simulink model "SoH_MPC_SolarPump"  (R2025b)
settings: Solver=ode4  StartTime=0.0  StopTime=86400  FixedStep=5  RelTol=1e-3
values from neighbouring files (symbols this model uses):
  P =     [robustness_same_min_tight.mat]    (also in robustness_same_min_wide.mat; run_day.m = rmfield(P, 'solverStep'); run_fixed_min.m = P0; P.strategy = 3; P.SoH0 = cases{k,2}; solver15_stress_check.m = mpc_params; P.strategy = strategy)
settings Model: Creator=Santhosh  LastModifiedBy=Santhosh

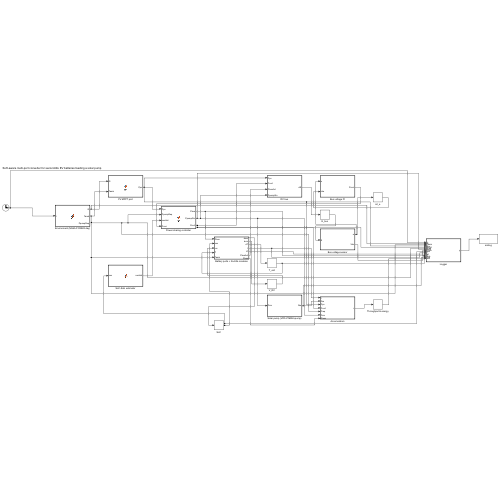
[thumbnail: Simulink's stored preview of the top-level diagram]
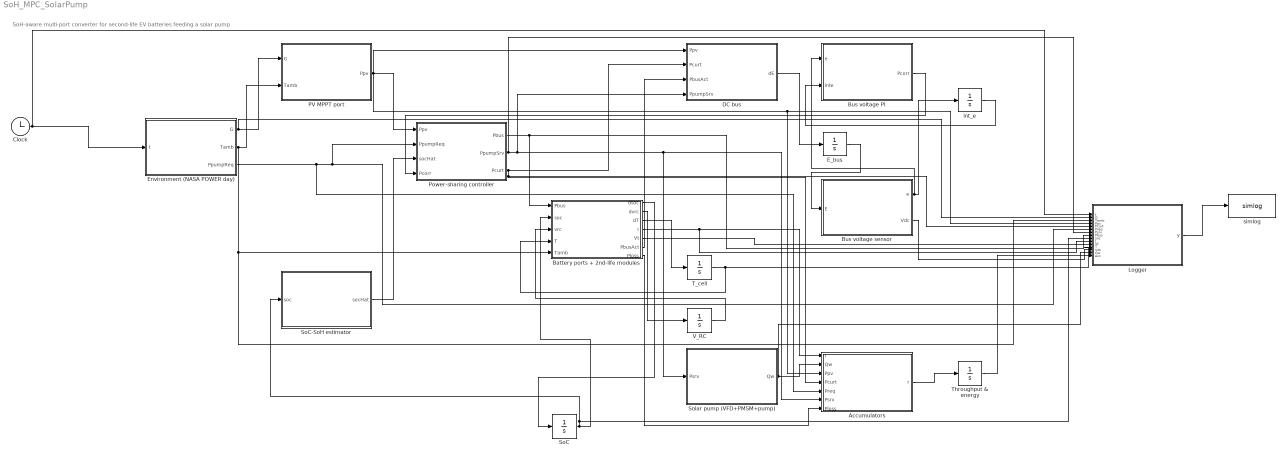
== system SoH_MPC_SolarPump ==
  note: SoH-aware multi-port converter for second-life EV batteries feeding a solar pump
  Accumulators : MATLAB Function  TreatAsAtomicUnit=on
  Battery ports + 2nd-life modules : MATLAB Function  TreatAsAtomicUnit=on
  Bus voltage PI : MATLAB Function  TreatAsAtomicUnit=on
  Bus voltage sensor : MATLAB Function  TreatAsAtomicUnit=on
  Clock : Clock
  DC bus : MATLAB Function  TreatAsAtomicUnit=on
  E_bus : Integrator  InitialCondition=P.Eref
  Environment (NASA POWER day) : MATLAB Function  TreatAsAtomicUnit=on
  Logger : MATLAB Function  TreatAsAtomicUnit=on
  PV MPPT port : MATLAB Function  TreatAsAtomicUnit=on
  Power-sharing controller : MATLAB Function  TreatAsAtomicUnit=on
  SoC : Integrator  InitialCondition=P.soc0
  SoC-SoH estimator : MATLAB Function  TreatAsAtomicUnit=on
  Solar pump (VFD+PMSM+pump) : MATLAB Function  TreatAsAtomicUnit=on
  T_cell : Integrator  InitialCondition=P.T0
  Throughput & energy : Integrator  InitialCondition=zeros(1,14)
  V_RC : Integrator  InitialCondition=zeros(1,4)
  int_e : Integrator  LimitOutput=on  UpperSaturationLimit=P.PcorrMax/P.Ki  LowerSaturationLimit=-P.PcorrMax/P.Ki
  simlog : ToWorkspace  VariableName=simlog  SampleTime=-1
      settings: Decimation=6
  wires:
  Clock/1 -> Environment (NASA POWER day)/1(t), Logger/1(t)
  Environment (NASA POWER day)/1(G) -> PV MPPT port/1(G), Logger/2(G)
  Environment (NASA POWER day)/2(Tamb) -> Battery ports + 2nd-life modules/5(Tamb), Logger/3(Tamb), PV MPPT port/2(Tamb)
  PV MPPT port/1(Ppv) -> Accumulators/3(Ppv), Logger/4(Ppv), Power-sharing controller/1(Ppv), DC bus/1(Ppv)
  Environment (NASA POWER day)/3(PpumpReq) -> Logger/6(Preq), Power-sharing controller/2(PpumpReq), Accumulators/5(Preq)
  SoC-SoH estimator/1(socHat) -> Power-sharing controller/3(socHat)
  Bus voltage PI/1(Pcorr) -> Power-sharing controller/4(Pcorr)
  Power-sharing controller/1(Pbus) -> Battery ports + 2nd-life modules/1(Pbus), Logger/8(Pbus)
  SoC/1 -> SoC-SoH estimator/1(soc), Logger/9(soc), Battery ports + 2nd-life modules/2(soc)
  V_RC/1 -> Battery ports + 2nd-life modules/3(vrc)
  T_cell/1 -> Battery ports + 2nd-life modules/4(T), Logger/12(T)
  Battery ports + 2nd-life modules/1(dsoc) -> SoC/1
  Battery ports + 2nd-life modules/2(dvrc) -> V_RC/1
  Battery ports + 2nd-life modules/3(dT) -> T_cell/1
  Power-sharing controller/3(Pcurt) -> Accumulators/4(Pcurt), Logger/5(Pcurt), DC bus/2(Pcurt)
  Battery ports + 2nd-life modules/6(PbusAct) -> DC bus/3(PbusAct)
  Power-sharing controller/2(PpumpSrv) -> Accumulators/6(Psrv), Solar pump (VFD+PMSM+pump)/1(Psrv), DC bus/4(PpumpSrv), Logger/7(Psrv)
  DC bus/1(dE) -> E_bus/1
  E_bus/1 -> Bus voltage sensor/1(E)
  Bus voltage sensor/1(e) -> int_e/1, Bus voltage PI/1(e)
  int_e/1 -> Bus voltage PI/2(inte)
  Battery ports + 2nd-life modules/4(I) -> Accumulators/1(I), Logger/10(I)
  Solar pump (VFD+PMSM+pump)/1(Qw) -> Accumulators/2(Qw), Logger/14(Qw)
  Battery ports + 2nd-life modules/7(Ploss) -> Accumulators/7(Ploss)
  Accumulators/1(r) -> Throughput & energy/1
  Battery ports + 2nd-life modules/5(Vt) -> Logger/11(Vt)
  Bus voltage sensor/2(Vdc) -> Logger/13(Vdc)
  Throughput & energy/1 -> Logger/15(acc)
  Logger/1(y) -> simlog/1

== matlab function SoH_MPC_SolarPump/Solar pump (VFD+PMSM+pump) ==
  data: Psrv input size=1; Qw output size=1; P parameter
function Qw = fcn(Psrv,P)
Qw = pump_model(Psrv,P);

== matlab function SoH_MPC_SolarPump/Accumulators ==
  data: I input size=[1 4]; r output size=[1 14]; Qw input size=1; Ppv input size=1; Pcurt input size=1; Preq input size=1; Psrv input size=1; Ploss input size=1
function r = fcn(I,Qw,Ppv,Pcurt,Preq,Psrv,Ploss)
r = [abs(I) max(I,0) Qw Ppv Pcurt Preq Psrv Ploss];

== matlab function SoH_MPC_SolarPump/Logger ==
  data: t input size=1; y output size=[1 43]; G input size=1; Tamb input size=1; Ppv input size=1; Pcurt input size=1; Preq input size=1; Psrv input size=1; Pbus input size=[1 4]; soc input size=[1 4]; I input size=[1 4]; Vt input size=[1 4]; T input size=[1 4]; Vdc input size=1; Qw input size=1; acc input size=[1 14]
function y = fcn(t,G,Tamb,Ppv,Pcurt,Preq,Psrv,Pbus,soc,I,Vt,T,Vdc,Qw,acc)
y = [t G Tamb Ppv Pcurt Preq Psrv Pbus soc I Vt T Vdc Qw acc];

== matlab function SoH_MPC_SolarPump/PV MPPT port ==
  data: G input size=1; Ppv output size=1; Tamb input size=1; P parameter
function Ppv = fcn(G,Tamb,P)
Ppv = pv_port(G,Tamb,P);

== matlab function SoH_MPC_SolarPump/Environment (NASA POWER day) ==
  data: t input size=1; G output size=1; Tamb output size=1; PpumpReq output size=1; P parameter
function [G,Tamb,PpumpReq] = fcn(t,P)
[G,Tamb,PpumpReq] = env_profile(t,P);

== matlab function SoH_MPC_SolarPump/SoC-SoH estimator ==
  data: soc input size=[1 4]; socHat output size=[1 4]; P parameter
function socHat = fcn(soc,P)
socHat = min(max(soc + P.socBias,0),1);

== matlab function SoH_MPC_SolarPump/Power-sharing controller ==
  data: Ppv input size=1; Pbus output size=[1 4]; PpumpReq input size=1; socHat input size=[1 4]; Pcorr input size=1; PpumpSrv output size=1; Pcurt output size=1; P parameter
function [Pbus,PpumpSrv,Pcurt] = fcn(Ppv,PpumpReq,socHat,Pcorr,P)
[Pbus,PpumpSrv,Pcurt] = share_ctrl(Ppv,PpumpReq,socHat,Pcorr,P);

== matlab function SoH_MPC_SolarPump/Battery ports + 2nd-life modules ==
  data: Pbus input size=[1 4]; dsoc output size=[1 4]; soc input size=[1 4]; vrc input size=[1 4]; T input size=[1 4]; Tamb input size=1; dvrc output size=[1 4]; dT output size=[1 4]; I output size=[1 4]; Vt output size=[1 4]; PbusAct output size=[1 4]; Ploss output size=1; P parameter
function [dsoc,dvrc,dT,I,Vt,PbusAct,Ploss] = fcn(Pbus,soc,vrc,T,Tamb,P)
[dsoc,dvrc,dT,I,Vt,PbusAct,Ploss] = batt_ports(Pbus,soc,vrc,T,Tamb,P);

== matlab function SoH_MPC_SolarPump/DC bus ==
  data: Ppv input size=1; dE output size=1; Pcurt input size=1; PbusAct input size=[1 4]; PpumpSrv input size=1
function dE = fcn(Ppv,Pcurt,PbusAct,PpumpSrv)
dE = Ppv - Pcurt + sum(PbusAct) - PpumpSrv;

== matlab function SoH_MPC_SolarPump/Bus voltage sensor ==
  data: E input size=1; e output size=1; Vdc output size=1; P parameter
function [e,Vdc] = fcn(E,P)
e = P.Eref - E;
Vdc = sqrt(2*max(E,0)/P.Cbus);

== matlab function SoH_MPC_SolarPump/Bus voltage PI ==
  data: e input size=1; Pcorr output size=1; inte input size=1; P parameter
function Pcorr = fcn(e,inte,P)
Pcorr = min(max(P.Kp*e + P.Ki*inte, -P.PcorrMax), P.PcorrMax);
